simulink model "launch_gate_exp"  (R2022b)
settings: Solver=FixedStepDiscrete  StartTime=0.0  StopTime=5  FixedStep=0.001  RelTol=1e-3
InitFcn:
  | if ~exist('P','var') || ~isfield(P,'gate_version'), P=gate_params(launch_tcs_params()); end
model workspace (MAT data in the model file):
  w_2 : Simulink.Parameter (value not decoded)
undefined symbols (not defined in the file): A, a, B, b, C, D, DiscIntNeverNeededParam, Iz, K, k1, K1, k2, K2, L1, L2, m, magnitude, Phi, Sample_time, Steer_Ratio
libraries: simulink x26, slpidlib x13, Solver_SF x1, dsparch4 x1
(part 6 of 7)

== matlab function launch_gate_exp/牵引效率计算/右前轮 ==
  data: Tw input; Fx_est output; omega_meas input; Fz input; Fx_raw output; Fx_limited output; omega_hat_out output; e_omega output; wv output
function [Fx_est, Fx_raw, Fx_limited, omega_hat_out, e_omega, wv] = ...
    FrontWheelFxObserver(Tw, omega_meas, Fz)

%#codegen
% 单轮纵向驱动力观测器
% 输入仅保留时变信号：
%   Tw         : 轮端驱动力矩 [N*m]
%   omega_meas : 实测车轮角速度 [rad/s]
%   Fz         : 单轮垂直载荷 [N]
%
% 输出：
%   Fx_est        : 最终纵向驱动力估计 [N]
%   Fx_raw        : 原始观测力估计 [N]
%   Fx_limited    : 限幅后力估计 [N]
%   omega_hat_out : 观测器内部估计轮速 [rad/s]
%   e_omega       : 轮速误差 [rad/s]
%   wv            : 低速平滑权重 [-]

% =========================================================
% 1. 固定参数区：根据具体车轮统一在这里调整
% =========================================================

Re = 0.834;              % 有效滚动半径 [m]
Jw = 110.64;            % 车轮等效转动惯量 [kg*m^2]
Ts = 0.001;             % 采样周期 [s]

mu = 0.7;               % 等效附着系数 [-]

l_omega = 50.0;         % 轮速误差反馈增益
fF = 3.0;               % 轮胎力观测带宽 [Hz]
gamma_F = Jw / Re * (2*pi*fF)^2;

enable_smc = 0;         % 是否启用滑模鲁棒项：1启用，0关闭
phi = 1.5;              % 滑模边界层厚度 [rad/s]
Func_ratio = 0.10;      % 未建模力比例，建议0.05~0.20
ks = Re / Jw * Func_ratio * mu * max(Fz, 0.0);

enable_lpf = 0;         % 是否启用输出低通：1启用，0关闭
tau_F = 0.08;           % 输出低通时间常数 [s]

v0 = 0.10;              % 低速权重起点 [m/s]
v1 = 0.80;              % 低速权重终点 [m/s]

eps_neg = 0.0;          % 允许负驱动力比例；严格驱动力估计取0
T_offset = 0.0;         % 轮端扭矩零偏 [N*m]
T_dead = 10.0;          % 扭矩死区 [N*m]

allow_brake_force = 0;  % 0：只估计驱动力；1：允许估计制动力

% =========================================================
% 2. 持久状态变量
% =========================================================

persistent omega_hat
persistent Fx_hat
persistent Fx_filt
persistent initialized

if isempty(initialized)
    omega_hat = 0.0;
    Fx_hat = 0.0;
    Fx_filt = 0.0;
    initialized = false;
end

if ~initialized
    omega_hat = omega_meas;
    Fx_hat = 0.0;
    Fx_filt = 0.0;
    initialized = true;
end

% =========================================================
% 3. 参数保护
% =========================================================

Jw_safe = max(Jw, 1e-6);
Re_safe = max(Re, 1e-6);
Ts_safe = max(Ts, 1e-6);
phi_safe = max(phi, 1e-6);
tau_safe = max(tau_F, Ts_safe);

Fz_safe = max(Fz, 0.0);
mu_safe = max(mu, 0.0);

if v1 <= v0
    v1_safe = v0 + 1e-3;
else
    v1_safe = v1;
end

% =========================================================
% 4. 扭矩零偏与死区处理
% =========================================================

Tw_corr = Tw - T_offset;

if abs(Tw_corr) < T_dead
    Tw_eff = 0.0;
else
    if Tw_corr > 0.0
        Tw_eff = Tw_corr - T_dead;
    else
        Tw_eff = Tw_corr + T_dead;
    end
end

if allow_brake_force < 0.5
    if Tw_eff < 0.0
        Tw_eff = 0.0;
    end
end

% =========================================================
% 5. 轮速误差
% =========================================================

e_omega = omega_meas - omega_hat;

% =========================================================
% 6. 滑模鲁棒项
% =========================================================

s = e_omega / phi_safe;

if s > 1.0
    sat_s = 1.0;
elseif s < -1.0
    sat_s = -1.0;
else
    sat_s = s;
end

if enable_smc > 0.5
    smc_term = ks * sat_s;
else
    smc_term = 0.0;
end

% =========================================================
% 7. 观测器状态更新
% =========================================================
%
% omega_hat_dot = Tw/Jw - Re/Jw*Fx_hat + l_omega*e_omega + ks*sat(e/phi)
% Fx_hat_dot    = -gamma_F*e_omega

omega_hat_dot = ...
    Tw_eff / Jw_safe ...
    - Re_safe / Jw_safe * Fx_hat ...
    + l_omega * e_omega ...
    + smc_term;

Fx_hat_dot = -gamma_F * e_omega;

omega_hat = omega_hat + Ts_safe * omega_hat_dot;
Fx_hat = Fx_hat + Ts_safe * Fx_hat_dot;

% =========================================================
% 8. 物理限幅与抗积分发散
% =========================================================

Fx_max = mu_safe * Fz_safe;

if allow_brake_force > 0.5
    Fx_min = -mu_safe * Fz_safe;
else
    Fx_min = -eps_neg * Fz_safe;
end

if Fx_hat > Fx_max
    Fx_hat = Fx_max;
elseif Fx_hat < Fx_min
    Fx_hat = Fx_min;
end

Fx_raw = Fx_hat;

if Fx_raw > Fx_max
    Fx_limited = Fx_max;
elseif Fx_raw < Fx_min
    Fx_limited = Fx_min;
else
    Fx_limited = Fx_raw;
end

% =========================================================
% 9. 低速平滑权重
% =========================================================

vw = abs(Re_safe * omega_meas);

wv = (vw - v0) / (v1_safe - v0);

if wv > 1.0
    wv = 1.0;
elseif wv < 0.0
    wv = 0.0;
end

wv = wv * wv * (3.0 - 2.0 * wv);

Fx_weighted = wv * Fx_limited;

% =========================================================
% 10. 输出低通滤波
% =========================================================

if enable_lpf > 0.5
    alpha = exp(-Ts_safe / tau_safe);
    Fx_filt = alpha * Fx_filt + (1.0 - alpha) * Fx_weighted;
    Fx_est = Fx_filt;
else
    Fx_filt = Fx_weighted;
    Fx_est = Fx_weighted;
end

omega_hat_out = omega_hat;

end

== matlab function launch_gate_exp/驱动防滑模块/MATLAB Function3 ==
  data: vfl input; v output; vfr input; vrl input; vrr input; omega input; brk input; st input
function v = fcn(vfl,vfr,vrl,vrr,omega,brk,st)
d = 2.36;
brk_bank = 40;
st_bank = 10;

v = 0;
if abs(st) <= st_bank && brk < brk_bank
    v = min([vfl,vfr,vrl,vrr]);
elseif abs(st) <= st_bank && brk >= brk_bank
    v = max([vfl,vfr,vrl,vrr]);
elseif abs(st) > st_bank && brk >= brk_bank
    v = 0.5*max([vfl+vrl-d*omega,vfr+vrr+d*omega]);
elseif abs(st) > st_bank && brk < brk_bank
    v = 0.5*max([vfl+vrl-d*omega,vfr+vrr+d*omega]);
end

== matlab function launch_gate_exp/牵引效率计算/左前轮 ==
  data: Tw input; Fx_est output; omega_meas input; Fz input; Fx_raw output; Fx_limited output; omega_hat_out output; e_omega output; wv output
function [Fx_est, Fx_raw, Fx_limited, omega_hat_out, e_omega, wv] = ...
    FrontWheelFxObserver(Tw, omega_meas, Fz)

%#codegen
% 单轮纵向驱动力观测器
% 输入仅保留时变信号：
%   Tw         : 轮端驱动力矩 [N*m]
%   omega_meas : 实测车轮角速度 [rad/s]
%   Fz         : 单轮垂直载荷 [N]
%
% 输出：
%   Fx_est        : 最终纵向驱动力估计 [N]
%   Fx_raw        : 原始观测力估计 [N]
%   Fx_limited    : 限幅后力估计 [N]
%   omega_hat_out : 观测器内部估计轮速 [rad/s]
%   e_omega       : 轮速误差 [rad/s]
%   wv            : 低速平滑权重 [-]

% =========================================================
% 1. 固定参数区：根据具体车轮统一在这里调整
% =========================================================

Re = 0.834;              % 有效滚动半径 [m]
Jw = 110.64;            % 车轮等效转动惯量 [kg*m^2]
Ts = 0.001;             % 采样周期 [s]

mu = 0.7;               % 等效附着系数 [-]

l_omega = 50.0;         % 轮速误差反馈增益
fF = 3.0;               % 轮胎力观测带宽 [Hz]
gamma_F = Jw / Re * (2*pi*fF)^2;

enable_smc = 0;         % 是否启用滑模鲁棒项：1启用，0关闭
phi = 1.5;              % 滑模边界层厚度 [rad/s]
Func_ratio = 0.10;      % 未建模力比例，建议0.05~0.20
ks = Re / Jw * Func_ratio * mu * max(Fz, 0.0);

enable_lpf = 0;         % 是否启用输出低通：1启用，0关闭
tau_F = 0.08;           % 输出低通时间常数 [s]

v0 = 0.10;              % 低速权重起点 [m/s]
v1 = 0.80;              % 低速权重终点 [m/s]

eps_neg = 0.0;          % 允许负驱动力比例；严格驱动力估计取0
T_offset = 0.0;         % 轮端扭矩零偏 [N*m]
T_dead = 10.0;          % 扭矩死区 [N*m]

allow_brake_force = 0;  % 0：只估计驱动力；1：允许估计制动力

% =========================================================
% 2. 持久状态变量
% =========================================================

persistent omega_hat
persistent Fx_hat
persistent Fx_filt
persistent initialized

if isempty(initialized)
    omega_hat = 0.0;
    Fx_hat = 0.0;
    Fx_filt = 0.0;
    initialized = false;
end

if ~initialized
    omega_hat = omega_meas;
    Fx_hat = 0.0;
    Fx_filt = 0.0;
    initialized = true;
end

% =========================================================
% 3. 参数保护
% =========================================================

Jw_safe = max(Jw, 1e-6);
Re_safe = max(Re, 1e-6);
Ts_safe = max(Ts, 1e-6);
phi_safe = max(phi, 1e-6);
tau_safe = max(tau_F, Ts_safe);

Fz_safe = max(Fz, 0.0);
mu_safe = max(mu, 0.0);

if v1 <= v0
    v1_safe = v0 + 1e-3;
else
    v1_safe = v1;
end

% =========================================================
% 4. 扭矩零偏与死区处理
% =========================================================

Tw_corr = Tw - T_offset;

if abs(Tw_corr) < T_dead
    Tw_eff = 0.0;
else
    if Tw_corr > 0.0
        Tw_eff = Tw_corr - T_dead;
    else
        Tw_eff = Tw_corr + T_dead;
    end
end

if allow_brake_force < 0.5
    if Tw_eff < 0.0
        Tw_eff = 0.0;
    end
end

% =========================================================
% 5. 轮速误差
% =========================================================

e_omega = omega_meas - omega_hat;

% =========================================================
% 6. 滑模鲁棒项
% =========================================================

s = e_omega / phi_safe;

if s > 1.0
    sat_s = 1.0;
elseif s < -1.0
    sat_s = -1.0;
else
    sat_s = s;
end

if enable_smc > 0.5
    smc_term = ks * sat_s;
else
    smc_term = 0.0;
end

% =========================================================
% 7. 观测器状态更新
% =========================================================
%
% omega_hat_dot = Tw/Jw - Re/Jw*Fx_hat + l_omega*e_omega + ks*sat(e/phi)
% Fx_hat_dot    = -gamma_F*e_omega

omega_hat_dot = ...
    Tw_eff / Jw_safe ...
    - Re_safe / Jw_safe * Fx_hat ...
    + l_omega * e_omega ...
    + smc_term;

Fx_hat_dot = -gamma_F * e_omega;

omega_hat = omega_hat + Ts_safe * omega_hat_dot;
Fx_hat = Fx_hat + Ts_safe * Fx_hat_dot;

% =========================================================
% 8. 物理限幅与抗积分发散
% =========================================================

Fx_max = mu_safe * Fz_safe;

if allow_brake_force > 0.5
    Fx_min = -mu_safe * Fz_safe;
else
    Fx_min = -eps_neg * Fz_safe;
end

if Fx_hat > Fx_max
    Fx_hat = Fx_max;
elseif Fx_hat < Fx_min
    Fx_hat = Fx_min;
end

Fx_raw = Fx_hat;

if Fx_raw > Fx_max
    Fx_limited = Fx_max;
elseif Fx_raw < Fx_min
    Fx_limited = Fx_min;
else
    Fx_limited = Fx_raw;
end

% =========================================================
% 9. 低速平滑权重
% =========================================================

vw = abs(Re_safe * omega_meas);

wv = (vw - v0) / (v1_safe - v0);

if wv > 1.0
    wv = 1.0;
elseif wv < 0.0
    wv = 0.0;
end

wv = wv * wv * (3.0 - 2.0 * wv);

Fx_weighted = wv * Fx_limited;

% =========================================================
% 10. 输出低通滤波
% =========================================================

if enable_lpf > 0.5
    alpha = exp(-Ts_safe / tau_safe);
    Fx_filt = alpha * Fx_filt + (1.0 - alpha) * Fx_weighted;
    Fx_est = Fx_filt;
else
    Fx_filt = Fx_weighted;
    Fx_est = Fx_weighted;
end

omega_hat_out = omega_hat;

end

== matlab function launch_gate_exp/质心侧偏角滑模观测器估计/Subsystem/MATLAB Function ==
  data: vx input; d_vy_model output; delta_f input; vy_hat input; gamma_hat input; d_gamma_model output
function [d_vy_model, d_gamma_model] = fcn(vx, delta_f, vy_hat, gamma_hat)

% 声明我们将使用来自MATLAB基础工作区的参数
m = 18530;%质量
Iz = 67536;%绕Z轴的转动惯量
a = 2.043;%前轴距
b=1.362;%后轴距
% Cf = 1360400;%前侧偏刚度
% Cr = 1611200;%后侧偏刚度
 Cf = 304828*2;Cr = 417040*2; % 仿真用

% 防止vx为0导致计算错误
if abs(vx) < 0.1
    vx = 0.1;
end

% 二自由度模型方程
d_vy_model = (-(Cf + Cr) / (m * vx)) * vy_hat + ...
             ((b * Cr - a * Cf) / (m * vx) - vx) * gamma_hat + ...
             (Cf / m) * delta_f;

d_gamma_model = ((b * Cr - a * Cf) / (Iz * vx)) * vy_hat - ...
                ((a^2 * Cf + b^2 * Cr) / (Iz * vx)) * gamma_hat + ...
                (a * Cf / Iz) * delta_f;

== matlab function launch_gate_exp/质心侧偏角滑模观测器估计/Subsystem1/MATLAB Function ==
  data: vx input; d_vy_model output; delta_f input; vy_hat input; gamma_hat input; d_gamma_model output
function [d_vy_model, d_gamma_model] = fcn(vx, delta_f, vy_hat, gamma_hat)

% 声明我们将使用来自MATLAB基础工作区的参数
m = 18530;%质量
Iz = 67536;%绕Z轴的转动惯量
a = 2.043;%前轴距
b=1.362;%后轴距
Cf = 1360400;%前侧偏刚度
Cr = 1611200;%后侧偏刚度

% 防止vx为0导致计算错误
if abs(vx) < 0.1
    vx = 0.1;
end

% 二自由度模型方程
d_vy_model = (-(Cf + Cr) / (m * vx)) * vy_hat + ...
             ((b * Cr - a * Cf) / (m * vx) - vx) * gamma_hat + ...
             (Cf / m) * delta_f;

d_gamma_model = ((b * Cr - a * Cf) / (Iz * vx)) * vy_hat - ...
                ((a^2 * Cf + b^2 * Cr) / (Iz * vx)) * gamma_hat + ...
                (a * Cf / Iz) * delta_f;

== matlab function launch_gate_exp/PF车速估计 ==
  data: ax_m input; vx_est output; ay_m input; r_m input; vy_est output; init_vx input; init_vy input
function [vx_est, vy_est] = fcn_ImprovedPF(ax_m, ay_m, r_m, init_vx, init_vy)
% 基于改进粒子滤波的车速估计
% 严格按照论文公式 (5)-(19) 实现

% --- 参数定义 (可根据实际情况调整) ---
persistent particles weights first_run
persistent T mx my mr Q R

if isempty(first_run)
    % 初始化参数
    N = 200; % 粒子数量 (论文伪代码步骤 0)
    T = 0.01; % 采样时间，对应传感器更新频率 (0.01s)
    
    % 自定义常数 (公式 17) - 需要根据调试确定
    mx = 0.5; 
    my = 0.5;
    mr = 0.1;
    
    % 过程噪声标准差 (公式 12 & 18) - 这里的 u 对应 xi
    sigma_proc = [0.1; 0.1; 0.01]; % [xi_x, xi_y, xi_z]
    Q = diag(sigma_proc.^2); 

    % 观测噪声标准差 (公式 13)
    sigma_meas = [0.2; 0.2; 0.01]; % [omega_ax, omega_ay, omega_r]
    R = diag(sigma_meas.^2);
    
    % --- 1. 初始化滤波器 (论文伪代码步骤 1) ---
    % 状态向量 X = [vx, ax, vy, ay, r]' (5维)
    % 粒子初始化：在初始值附近添加随机扰动
    particles = zeros(5, N);
    particles(1, :) = init_vx + randn(1, N) * 0.5; % vx
    particles(2, :) = ax_m + randn(1, N) * 0.1;    % ax
    particles(3, :) = init_vy + randn(1, N) * 0.1; % vy
    particles(4, :) = ay_m + randn(1, N) * 0.1;    % ay
    particles(5, :) = r_m + randn(1, N) * 0.01;    % r
    
    weights = ones(1, N) / N; % 初始化权重
    
    first_run = 0;
end

N = size(particles, 2);
particles_next = zeros(5, N);

% 测量向量 Z_k (公式 13上方定义)
Z_k = [ax_m; ay_m; r_m]; 

% --- 2. 粒子滤波主循环 ---
% 对应论文伪代码的步骤 2-8 (针对每个时刻)

% 预计算 G 矩阵的一部分 (公式 11) 和 L 矩阵的一部分 (公式 17)
% 注意：G 和 L 实际上在每个粒子计算中略有不同吗？
% 论文中 G 是常数矩阵，但 L 取决于测量值与上一时刻状态的差，
% 且公式 (19) X_k = F*X_k-1 + P_k + G*L*xi
% 这里我们需要对每个粒子进行循环

for i = 1:N
    % 提取第 i 个粒子上一时刻的状态 X_k-1
    X_prev = particles(:, i);
    vx_prev = X_prev(1);
    ax_prev = X_prev(2);
    vy_prev = X_prev(3);
    ay_prev = X_prev(4);
    r_prev  = X_prev(5);
    
    % --- 计算状态转移矩阵 F_k (公式 10) ---
    % 注意：原论文公式(10)中有笔误，第二行和第四行应该是全0行还是保持加速度不变？
    % 通常 CA (Constant Acceleration) 模型加速度导数为0。
    % 论文公式(10) F_k 矩阵：
    % Row 1: vx = vx + ax*T + vy*r*T (源自 ax = vx_dot - vy*r -> vx_dot = ax + vy*r) -> 离散化: vx_k = vx_k-1 + ax_k-1*T + vy_k-1*r_k-1*T (对应公式 7)
    % Row 2: ax = ax (常数模型) -> 0 1 0 0 0
    % Row 3: vy = vy + ay*T - vx*r*T (源自 ay = vy_dot + vx*r -> vy_dot = ay - vx*r) -> 离散化: vy_k = vy_k-1 + ay_k-1*T - vx_k-1*r_k-1*T (对应公式 8)
    % Row 4: ay = ay -> 0 0 0 1 0
    % Row 5: r = r -> 0 0 0 0 1
    
    F_k = [1, T,  r_prev*T, 0, 0;
           0, 1,         0, 0, 0;
          -r_prev*T, 0,  1, T, 0;
           0, 0,         0, 1, 0;
           0, 0,         0, 0, 1];
       
    % --- 3. 计算提议分布修正项 P_k (公式 14) ---
    % 论文中 a_x,k-1 是粒子状态，而 Z 中的 a_x 是当前测量值。
    % 公式 (14) 利用了测量值与粒子状态的差值。
    % 注意下标：公式里用的是 k-1 时刻的测量值和粒子，但在实时运行中，我们通常拿当前测量值去修正预测。
    % 也就是论文提到的 "基于 k-1 时刻传感器测量值...与 k-1 时刻每个粒子的...差值"。
    % 这里为了代码简洁，假设输入的 ax_m 即为 k-1 时刻（或者当前时刻用来修正前一步）。
    % 严格照公式：
    diff_ax = ax_m - ax_prev; % (a_xz,k-1 - a^i_x,k-1)
    diff_ay = ay_m - ay_prev; % (a_yz,k-1 - a^i_y,k-1)
    diff_r  = r_m  - r_prev;  % (r_z,k-1 - r^i_k-1)
    
    P_k = [T * (diff_ax + diff_r); % 第一行对应 vx 的修正
           diff_ax;                % 第二行对应 ax 的修正
           T * (diff_ay + diff_r); % 第三行对应 vy 的修正
           diff_ay;                % 第四行对应 ay 的修正
           diff_r];                % 第五行对应 r  的修正
           
    % --- 计算自适应增益矩阵 L_k (公式 17) ---
    L_k = [mx * diff_ax, 0, 0;
           0, my * diff_ay, 0;
           0, 0, mr * diff_r];
       
    % --- 计算过程噪声矩阵 G (公式 11) ---
    G = [T^2/2, 0, 0;
         T,     0, 0;
         0, T^2/2, 0;
         0, T,     0;
         0, 0,     T];
         
    % --- 生成标准高斯噪声 xi (公式 18) ---
    % xi 对应伪代码中的 "相互独立的标准高斯噪声"
    xi = randn(3, 1); 
    
    % --- 4. 状态预测 (公式 19) ---
    % X_k = F_k * X_k-1 + P_k + G * L_k * xi
    particles_next(:, i) = F_k * X_prev + P_k + G * L_k * xi;
    
    % --- 5. 权重更新 (伪代码步骤 6 & 7) ---
    % 计算该粒子的预测观测值 Z_pre (公式 13)
    % Z = [ax, ay, r]'
    % 状态向量 X = [vx, ax, vy, ay, r]' -> 对应的索引是 2, 4, 5
    Z_pre = [particles_next(2, i); 
             particles_next(4, i); 
             particles_next(5, i)];
         
    % 计算似然 (高斯分布)
    % likelihood = (1/sqrt((2*pi)^3 * det(R))) * exp(-0.5 * (Z_k - Z_pre)' * inv(R) * (Z_k - Z_pre));
    % 简化计算 (忽略常数项，因为最后会归一化)
    error = Z_k - Z_pre;
    likelihood = exp(-0.5 * (error' / R * error));
    
    weights(i) = weights(i) * likelihood;
end

% --- 6. 权重归一化 (伪代码步骤 10) ---
sum_weights = sum(weights);
if sum_weights > 0
    weights = weights / sum_weights;
else
    weights = ones(1, N) / N; % 防止除以零
end

% --- 7. 重采样 (伪代码步骤 9) ---
% 有效粒子数 (N_eff) 判断是否需要重采样
N_eff = 1 / sum(weights.^2);
if N_eff < N / 2
    particles_next = Resample(particles_next, weights, N);
    weights = ones(1, N) / N;
end

% 更新粒子集
particles = particles_next;

% --- 8. 输出状态估计 (伪代码步骤 11) ---
% 加权平均
vx_est = sum(particles(1, :) .* weights);
vy_est = sum(particles(3, :) .* weights);

end

% --- 辅助函数：重采样 (Systematic Resampling) ---
function new_particles = Resample(particles, weights, N)
    cdf = cumsum(weights);
    new_particles = zeros(size(particles));
    u = rand / N;
    j = 1;
    for i = 1:N
        u_i = u + (i - 1) / N;
        while u_i > cdf(j)
            j = j + 1;
            if j > N, j = N; end
        end
        new_particles(:, i) = particles(:, j);
    end
end

== matlab function launch_gate_exp/加速度滑模观测/MATLAB Function ==
  data: gamma_m input; phi_est output; phi_GPS input; GPS_valid input; gamma_corrected output; e_gamma_est output
function [phi_est, gamma_corrected, e_gamma_est] = GPS_INS_SlidingMode(gamma_m, phi_GPS, GPS_valid)
%% GPS/INS融合 - 滑模观测器
% 输入:
%   gamma_m   - INS测量的横摆角速度 (rad/s)
%   phi_GPS   - GPS测量的航向角 (rad)
%   GPS_valid - GPS数据有效标志
% 输出:
%   phi_est         - 估计的航向角 (rad)
%   gamma_corrected - 校正后的横摆角速度 (rad/s)
%   e_gamma_est     - 估计的横摆角速度偏差 (rad/s)

%% 参数设置
persistent phi_hat e_gamma_hat phi_GPS_last initialized

dt_sim = 0.001;      % 仿真步长 (s)

% ===== 滑模增益（主要调参对象）=====
k1 = 5;              % 航向角校正增益
k2 = 0.5;            % 角速度偏差校正增益
lambda = 10;         % 滑模面斜率

% 边界层厚度（消除抖振）
epsilon = 0.01;      % 越小越精确，但抖振越大

%% 初始化
if isempty(initialized)
    phi_hat = 0;
    e_gamma_hat = 0;
    phi_GPS_last = 0;
    initialized = true;
end

%% 滑模观测器核心算法

% 状态方程：
% phi_dot = gamma_m - e_gamma（真实角速度 = 测量值 - 偏差）
% e_gamma_dot ≈ 0（偏差缓慢变化）

if GPS_valid
    % 滑模面：s = phi_GPS - phi_hat
    s = phi_GPS - phi_hat;
    
    % 饱和函数（替代sign函数，减少抖振）
    if abs(s) > epsilon
        sat_s = sign(s);
    else
        sat_s = s / epsilon;
    end
    
    % 滑模观测器方程
    % 航向角估计
    phi_hat_dot = (gamma_m - e_gamma_hat) + k1 * sat_s;
    
    % 角速度偏差估计（利用滑模的等效控制）
    e_gamma_hat_dot = -k2 * sat_s;
    
    % 积分更新
    phi_hat = phi_hat + phi_hat_dot * dt_sim;
    e_gamma_hat = e_gamma_hat + e_gamma_hat_dot * dt_sim;
    
    % 保存GPS值
    phi_GPS_last = phi_GPS;
    
else
    % GPS无效时，纯惯性推算
    phi_hat = phi_hat + (gamma_m - e_gamma_hat) * dt_sim;
    % e_gamma_hat 保持不变
end

%% 输出
phi_est = phi_hat;
e_gamma_est = e_gamma_hat;
gamma_corrected = gamma_m - e_gamma_hat;

end

== matlab function launch_gate_exp/加速度滑模观测/MATLAB Function1 ==
  data: a_xm input; a_xc output; a_ym input; v_xGPS input; v_yGPS input; gamma_c input; GPS_update_flag input; a_yc output; e_ax_est output; e_ay_est output; reset input
function [a_xc, a_yc, e_ax_est, e_ay_est] = accel_SMO_correction(a_xm, a_ym, v_xGPS, v_yGPS, gamma_c, GPS_update_flag, reset)
% 加速度滑模观测器校正
% 输入：
%   a_xm, a_ym      - INS测量的加速度 (m/s^2)
%   v_xGPS, v_yGPS  - GPS测量的速度 (m/s)
%   gamma_c         - 校正后的横摆角速度 (rad/s)
%   GPS_update_flag - GPS更新标志 (1=有新数据)
%   reset           - 复位信号
% 输出：
%   a_xc, a_yc      - 校正后的加速度
%   e_ax_est, e_ay_est - 估计的加速度偏差

% 采样时间
dt = 0.001;     % 仿真步长
DT = 0.05;      % GPS采样周期

% 滑模观测器增益（需根据实际调参）
persistent k1 k2 lambda1 lambda2
if isempty(k1)
    k1 = 5;       % 速度误差增益
    k2 = 5;
    lambda1 = 0.5; % 加速度偏差增益
    lambda2 = 0.5;
end

% 持久变量（状态记忆）
persistent v_xI v_yI e_ax e_ay initialized
persistent a_xm_sum a_ym_sum sum_count

if isempty(initialized) || reset
    v_xI = 0;      % INS积分速度 x
    v_yI = 0;      % INS积分速度 y
    e_ax = 0;      % 加速度偏差估计 x
    e_ay = 0;      % 加速度偏差估计 y
    a_xm_sum = 0;  % 加速度累加（用于GPS周期内求和）
    a_ym_sum = 0;
    sum_count = 0;
    initialized = true;
end

% 累加加速度（对应论文中的求和项）
a_xm_sum = a_xm_sum + a_xm;
a_ym_sum = a_ym_sum + a_ym;
sum_count = sum_count + 1;

% 速度积分（考虑横摆角速度耦合，对应式3-10）
% v_xI(k+1) = v_xI(k) + dt*a_xm + DT*(v_yI*gamma_c - e_ax - n_ax)
% 简化：每步用校正后的加速度积分
a_xc_temp = a_xm - e_ax;
a_yc_temp = a_ym - e_ay;

% 考虑横摆角速度耦合的速度更新
v_xI = v_xI + dt * (a_xc_temp + v_yI * gamma_c);
v_yI = v_yI + dt * (a_yc_temp - v_xI * gamma_c);

% GPS更新时刻：执行滑模校正
if GPS_update_flag == 1
    % 速度误差（观测残差）
    e_vx = v_xI - v_xGPS;
    e_vy = v_yI - v_yGPS;
    
    % 滑模切换函数
    s_x = sign(e_vx);
    s_y = sign(e_vy);
    
    % 也可用饱和函数避免抖振
    % epsilon = 0.1;
    % s_x = sat_func(e_vx, epsilon);
    % s_y = sat_func(e_vy, epsilon);
    
    % 速度校正（直接用GPS速度重置，或软校正）
    % 软校正方式：
    v_xI = v_xI - k1 * DT * s_x;
    v_yI = v_yI - k2 * DT * s_y;
    
    % 加速度偏差更新（滑模观测器核心）
    e_ax = e_ax + lambda1 * DT * s_x;
    e_ay = e_ay + lambda2 * DT * s_y;
    
    % 限幅防止发散
    e_ax = max(min(e_ax, 2), -2);
    e_ay = max(min(e_ay, 2), -2);
    
    % 清零累加器
    a_xm_sum = 0;
    a_ym_sum = 0;
    sum_count = 0;
end

% 输出校正后的加速度（式3-12）
a_xc = a_xm - e_ax;
a_yc = a_ym - e_ay;

% 输出偏差估计（用于调试）
e_ax_est = e_ax;
e_ay_est = e_ay;

end

% 饱和函数（可选，减少抖振）
function y = sat_func(x, epsilon)
    if abs(x) <= epsilon
        y = x / epsilon;
    else
        y = sign(x);
    end
end

== matlab function launch_gate_exp/质心侧偏角观测/MATLAB Function ==
  data: x_hat input; x_dot output; u input; z_meas input; z_hat output
function [x_dot, z_hat] = fcn(x_hat, u, z_meas)

    % === 车辆物理参数 ===
    mv = 18530;       % Vehicle total mass (kg)
    Izz = 67536;      % Second moment of mass (kg m^2)
    L1 = 2.043;        % CG to front axle (m)
    L2 = 1.362;        % CG to rear axle (m)
    Cf1 = 304828 * 2;     % Front cornering stiffness (N/rad) - 对应图中 C_F\delta^1
    Cf2 = 417040 * 2;     % Rear cornering stiffness (N/rad) - 对应图中 C_F\delta^2

    % === 观测器参数===
    Lambda = [100, 0;    % 增益矩阵 (3x2)
          0, 100;    
          0, 1000];   
    lambda_param = 1;
    Ts = 0.001;           % 离散采样时间 (Discrete Sample Time)

    % === 1. 解包状态变量和输入 ===
    % x_hat = [Vg_est; delta_est; r_est] 
    x1 = x_hat(1); % V_G
    x2 = x_hat(2); % delta (侧偏角)
    x3 = x_hat(3); % psi_dot (横摆角速度)

    % u = [beta; Fl1; Fl2]
    u1 = u(1); % beta
    u2 = u(2); % Fl1
    u3 = u(3); % Fl2
    
    % 防止分母为0
    if abs(x1) < 0.1
        x1 = 0.1; 
    end

    % === 2. 计算估计的输出 z_hat  ===
    % z = [Vg; psi_dot]
    h_NL = [x1; x3]; 
    z_hat = h_NL;

    % === 3. 计算观测误差 (z - z_hat) ===
    error = z_meas - z_hat;

    % === 4. 计算 Sign_eq 函数 ===
    sign_term = (2/pi) * atan(lambda_param * error);

    % === 5. 计算非线性函数 ===
    term1_1 = (1/mv) * (u2 * cos(x2 - u1) + u3 * cos(x2));
    term1_2 = (1/mv) * Cf2 * (-x2 + L2*x3/x1) * sin(x2);
    term1_3 = (1/mv) * Cf1 * (u1 - x2 - L1*x3/x1) * sin(x2 - u1);
    
    dx1_val = term1_1 + term1_2 + term1_3;

    term2_1 = 1/(mv*x1) * (u2 * sin(u1 - x2) - u3 * sin(x2)) ;
    term2_2 = 1/(mv*x1) * Cf1 * (u1 - x2 - L1*x3/x1) * cos(u1 - x2);
    term2_3 = 1/(mv*x1) * Cf2 * (-x2 + L2*x3/x1) * cos(x2) - x3;
    
    dx2_val = term2_1 + term2_2 + term2_3;

    term3_1 = (1/Izz) * ( L1 * u2 * sin(u1) - L2 * Cf2 * (-x2 + L2*x3/x1) ); 
    term3_2 = (1/Izz) * L1 * Cf1 * (u1 - x2 - L1*x3/x1) * cos(u1);
    
    dx3_val = term3_1 + term3_2;
    
    f_NL = [dx1_val; dx2_val; dx3_val];

    % === 6. 最终观测器状态导数 ===
    % x_hat_dot = f_NL(x_hat, u) + Lambda * sign_eq(z - z_hat)
    x_dot = f_NL + Lambda * sign_term;
end

== matlab function launch_gate_exp/软土扭矩分配/牵引功率目标计算 ==
  data: dt_s input; drawbar_power_w output; wheel_omegas_radps input; previous_applied_torques_n_m input; longitudinal_speed_mps input; implement_force_x_n input; wheel_power_w output; phi_raw output; filtered_phi output; filtered_normalized_phi output; lambda_est output; objective_valid output
function [drawbar_power_w, wheel_power_w, phi_raw, filtered_phi, filtered_normalized_phi, lambda_est, objective_valid] = MF_TractionEfficiencyObjective(dt_s, wheel_omegas_radps, previous_applied_torques_n_m, longitudinal_speed_mps, implement_force_x_n)

% 牵引效率目标函数计算模块
%
% 本模块计算牵引效率相关的在线优化目标：
% eta = P_drawbar / P_wheel
%
% 并构造 Dinkelbach 差值型目标：
% phi = P_drawbar - lambda * P_wheel

persistent has_filtered_power filtered_drawbar_power_state filtered_wheel_power_state
persistent has_filtered_phi filtered_phi_state filtered_normalized_phi_state
persistent lambda_state

if isempty(has_filtered_power)

    has_filtered_power = 0.0;
    filtered_drawbar_power_state = 0.0;
    filtered_wheel_power_state = 0.0;

    has_filtered_phi = 0.0;
    filtered_phi_state = 0.0;
    filtered_normalized_phi_state = 0.0;

    lambda_state = 0.0;
end

%% 输入整理

dt = max(double(dt_s), 0.0);
omegas = row4_local(wheel_omegas_radps);
applied_torques = row4_local(previous_applied_torques_n_m);

vx = double(longitudinal_speed_mps);
implement_force = double(implement_force_x_n);

%% 轮端输入功率计算

% 轮端输入功率 P_wheel = sum(T_i * omega_i)。
% 只保留非负驱动功率，避免制动功率或异常信号影响牵引效率评价。
wheel_drive_powers = zeros(1, 4);

for index = 1:4
    wheel_drive_powers(index) = max(0.0, applied_torques(index) * abs(omegas(index)));
end

wheel_power_w = sum(wheel_drive_powers);

%% 有效牵引功率计算

% 农具阻力方向通常与车辆行驶方向相反。
% 前进时，如果 implement_force 为负，则 -implement_force 为有效牵引阻力。
% 倒车时符号相反。
if vx > 0.08
    drawbar_force = max(0.0, -implement_force);
elseif vx < -0.08
    drawbar_force = max(0.0, implement_force);
else
    drawbar_force = 0.0;
end

drawbar_power_w = drawbar_force * abs(vx);

%% 目标函数有效性判断

% 轮端输入功率过低或车速过低时，牵引效率计算不可靠。
objective_valid = wheel_power_w >= 100.0 && abs(vx) > 0.08;

%% 功率滤波

alpha_objective = first_order_alpha_local(dt, 0.7);

if has_filtered_power <= 0.5 || ~objective_valid

    filtered_drawbar_power_state = drawbar_power_w;
    filtered_wheel_power_state = wheel_power_w;
    has_filtered_power = 1.0;

else

    filtered_drawbar_power_state = filtered_drawbar_power_state + ...
        alpha_objective * (drawbar_power_w - filtered_drawbar_power_state);

    filtered_wheel_power_state = filtered_wheel_power_state + ...
        alpha_objective * (wheel_power_w - filtered_wheel_power_state);

    has_filtered_power = 1.0;
end

%% lambda 牵引效率参数更新

if objective_valid

    eta_instant = drawbar_power_w / max(wheel_power_w, 1.0e-9);

    alpha_lambda = first_order_alpha_local(dt, 1.0);

    lambda_state = lambda_state + alpha_lambda * (eta_instant - lambda_state);
end

lambda_est = lambda_state;

%% Dinkelbach 差值型性能指标

phi_raw = drawbar_power_w - lambda_est * wheel_power_w;

% 归一化性能指标，用于降低功率量级变化对极值寻优的影响。
normalized_phi = phi_raw / max(abs(wheel_power_w), 1000.0);

%% 性能指标滤波

if has_filtered_phi <= 0.5 || ~objective_valid

    filtered_phi_state = phi_raw;
    filtered_normalized_phi_state = normalized_phi;
    has_filtered_phi = 1.0;

else

    filtered_phi_state = filtered_phi_state + ...
        alpha_objective * (phi_raw - filtered_phi_state);

    filtered_normalized_phi_state = filtered_normalized_phi_state + ...
        alpha_objective * (normalized_phi - filtered_normalized_phi_state);

    has_filtered_phi = 1.0;
end

filtered_phi = filtered_phi_state;
filtered_normalized_phi = filtered_normalized_phi_state;

end


function output = row4_local(values)

% 将输入信号整理为 1×4 行向量。

input_values = double(values);
output = zeros(1, 4);

for index = 1:4
    output(index) = input_values(index);
end

end


function alpha = first_order_alpha_local(dt, time_constant_s)

% 一阶低通滤波系数：
% y(k) = y(k-1) + alpha * [u(k) - y(k-1)]

if dt <= 0.0 || time_constant_s <= 0.0
    alpha = 1.0;
else
    alpha = dt / (time_constant_s + dt);
end

end

== matlab function launch_gate_exp/软土扭矩分配/四轮目标滑移率计算 ==
  data: current_time_s input; adaptive_targets output; dt_s input; filtered_normalized_phi input; objective_valid input; kappa_valid input; target_base_out output; gradient_estimates output
function [adaptive_targets, target_base_out, gradient_estimates] = MF_AdaptiveSlipTarget4W(current_time_s, dt_s, filtered_normalized_phi, objective_valid, kappa_valid)

% 四轮自适应目标滑移率生成模块
%
% 采用多变量极值寻优思想，对四个车轮的目标滑移率进行独立更新。
%
% 四轮顺序：
% 1：左前轮
% 2：右前轮
% 3：左后轮
% 4：右后轮

persistent target_base_state gradient_state

if isempty(target_base_state)

    % 初始目标滑移率仍保持原前后轴标定值。
    target_base_state = [0.078, 0.078, 0.128, 0.128];

    % 四轮梯度估计初值。
    gradient_state = zeros(1, 4);
end

%% 输入整理

time_s = double(current_time_s);
dt = max(double(dt_s), 0.0);
normalized_phi = double(filtered_normalized_phi);
valid_vec = row4_local(kappa_valid);

%% 极值寻优参数

% 四轮扰动频率，单位 Hz。
frequencies = [0.7, 0.9, 1.1, 1.3];

% 目标滑移率扰动幅值。
perturb_amp = 0.002;

% 目标滑移率基值自适应增益。
adapt_gain = 0.0006;

% 目标滑移率允许范围。
target_min = 0.03;
target_max = 0.25;

% 梯度低通滤波系数。
alpha_gradient = first_order_alpha_local(dt, 0.8);

%% 是否允许更新目标基值

update_enabled = double(objective_valid) > 0.5 && all(valid_vec > 0.5);

%% 生成四轮扰动信号

sine_signals = zeros(1, 4);

for index = 1:4
    sine_signals(index) = sin(2.0 * pi * frequencies(index) * time_s);
end

%% 梯度估计与目标基值更新

if update_enabled

    for index = 1:4

        % 极值寻优解调。
        % 性能指标与扰动信号相乘，用于估计该轮目标滑移率变化对牵引效率目标的边际影响。
        gradient_raw = 2.0 * normalized_phi * sine_signals(index) / perturb_amp;

        % 梯度估计低通滤波。
        gradient_state(index) = gradient_state(index) + ...
            alpha_gradient * (gradient_raw - gradient_state(index));

        % 限制每个采样周期目标滑移率基值的最大变化量。
        max_delta = 0.003 * dt;

        target_delta = clamp_local(adapt_gain * gradient_state(index) * dt, -max_delta, max_delta);

        % 更新目标滑移率基值。
        target_base_state(index) = clamp_local(target_base_state(index) + target_delta, target_min, target_max);
    end
end

%% 输出四轮目标滑移率

adaptive_targets = zeros(1, 4);

for index = 1:4

    % 最终目标 = 基值 + 小幅正弦扰动。
    adaptive_targets(index) = clamp_local( ...
        target_base_state(index) + perturb_amp * sine_signals(index), ...
        target_min, target_max);
end

% 调试输出，可在 Simulink 中不连接。
target_base_out = target_base_state;
gradient_estimates = gradient_state;

end


function output = row4_local(values)

% 将输入信号整理为 1×4 行向量。

input_values = double(values);
output = zeros(1, 4);

for index = 1:4
    output(index) = input_values(index);
end

end


function alpha = first_order_alpha_local(dt, time_constant_s)

% 一阶低通滤波系数。

if dt <= 0.0 || time_constant_s <= 0.0
    alpha = 1.0;
else
    alpha = dt / (time_constant_s + dt);
end

end


function value = clamp_local(value_in, lower, upper)

% 数值限幅函数。

value = min(max(double(value_in), double(lower)), double(upper));

end

== matlab function launch_gate_exp/牵引效率计算/计算平均边际贡献 ==
  data: v_all input; phi output
function phi = shapley_calc(v_all)

% 输入:
% v_all: 16x1
%
% 子集顺序:
%
% 1  -> []
% 2  -> [1]
% 3  -> [2]
% 4  -> [3]
% 5  -> [4]
% 6  -> [1 2]
% 7  -> [1 3]
% 8  -> [1 4]
% 9  -> [2 3]
% 10 -> [2 4]
% 11 -> [3 4]
% 12 -> [1 2 3]
% 13 -> [1 2 4]
% 14 -> [1 3 4]
% 15 -> [2 3 4]
% 16 -> [1 2 3 4]
%
% 输出:
% phi = [FL; FR; RL; RR]

%% 平移法消除负值

v_min = min(v_all);

if v_min < 0
    v_all = v_all - v_min;
end

%% 参数

n = 4;

fact = factorial(0:n);

phi = zeros(4,1);

%% 联盟定义

coalitions = [...
    0 0 0 0;  % 1
    1 0 0 0;  % 2
    0 1 0 0;  % 3
    0 0 1 0;  % 4
    0 0 0 1;  % 5
    1 1 0 0;  % 6
    1 0 1 0;  % 7
    1 0 0 1;  % 8
    0 1 1 0;  % 9
    0 1 0 1;  % 10
    0 0 1 1;  % 11
    1 1 1 0;  % 12
    1 1 0 1;  % 13
    1 0 1 1;  % 14
    0 1 1 1;  % 15
    1 1 1 1]; % 16

%% Shapley计算

for i = 1:n

    for idx = 1:16

        S = coalitions(idx,:);

        % 若联盟中已有玩家i
        if S(i) == 1
            continue;
        end

        % 联盟大小
        k = sum(S);

        % 权重
        w = fact(k+1) * fact(n-k) / fact(n+1);

        % v(S)
        v_S = v_all(idx);

        % 构造 S∪{i}
        S_with_i = S;
        S_with_i(i) = 1;

        %% 查找 S∪{i} 对应索引

        idx_Si = 1;

        for j = 1:16

            if isequal(coalitions(j,:), S_with_i)

                idx_Si = j;
                break;

            end

        end

        % v(S∪{i})
        v_Si = v_all(idx_Si);

        % Shapley累加
        phi(i) = phi(i) + w * (v_Si - v_S);

    end

end

phi_min = min(phi);

if phi_min < 0
    phi = phi - phi_min;
end

end

== matlab function launch_gate_exp/协同博弈扭矩分配/MATLAB Function ==
  data: v input; alpha output
function alpha = fcn(v)

if v < 0.5
    alpha = 0;
elseif v < 5
    alpha = (v - 0.5)/(5 - 0.5);
else
    alpha = 1;
end

== matlab function launch_gate_exp/牵引效率计算/MATLAB Function3 ==
  data: Fx input; V_all output; Vx input; T input; uF input; mu input; Fz input; slip input; Mz_ref input; Traction_all output; lamdaN_all output; lamda_all output; Mz_all output
function [V_all,Traction_all,lamdaN_all,lamda_all,Mz_all] = shapley_value_all(...
Fx,...
Vx,...
T,...
uF,...
mu,...
Fz,...
slip,...
Mz_ref)

%% 参数

kf = 3;   % 前轮牵引权重
kr = 6;   % 后轮牵引权重

w1 = 100000;  % 滑转率损失权重
w2 = 5000;    % 附着利用率均衡权重
w3 = 0.0001;  % 横摆稳定损失权重

% 半轮距
bf = 2.39/2;
br = 2.33/2;

%% 初始化

V_all = zeros(16,1);
Traction_all = zeros(16,1);
lamdaN_all = zeros(16,1);
lamda_all = zeros(16,1);
Mz_all = zeros(16,1);

%% 16个联盟

coalitions = [...
    0 0 0 0;  % 空集-1
    1 0 0 0;  % 2
    0 1 0 0;  % 3
    0 0 1 0;  % 4
    0 0 0 1;  % 5
    1 1 0 0;  % 6
    1 0 1 0;  % 7
    1 0 0 1;  % 8
    0 1 1 0;  % 9
    0 1 0 1;  % 10
    0 0 1 1;  % 11
    1 1 1 0;  % 12
    1 1 0 1;  % 13
    1 0 1 1;  % 14
    0 1 1 1;  % 15
    1 1 1 1];  % 16

%% 遍历所有联盟

for k = 1:16

    coalition = coalitions(k,:)';

    %% 联盟数据

    Fx_s    = Fx    .* coalition;
    T_s     = T     .* coalition;
    uF_s    = uF   .* coalition;
    mu_s    = mu    .* coalition;
    Fz_s    = Fz    .* coalition;
    slip_s  = slip   .* coalition;

    %% 1 牵引能力项

    F_front = uF_s(1) + uF_s(2);
    F_rear  = uF_s(3) + uF_s(4);

    traction_term = ...
        kf * F_front + ...
        kr * F_rear;

    %% 2 滑转率损失

    
    % 只保留联盟中的驱动轮滑转率
    slip_active = abs(slip_s);

    % 防止空集导致 max([]) 问题
if sum(coalition) == 0

    lamdaN = 0;

else

    % 最大滑转率
    slip_max = max(slip_active);

    % 四次方强化惩罚
    lamdaN = slip_max^4;

end


    %% 3 附着利用率

    lambda_term = 0;

    for i = 1:4

        if coalition(i) == 1

            denom = uF_s(i);

            if abs(denom) > 1e-6

                lambda_i = Fx_s(i) / denom;

                % 平方强化
                lambda_term = ...
                    lambda_term + lambda_i^2;

            end

        end

    end

    %% 4 横摆力矩

    Mz = ...
        (-Fx_s(1) + Fx_s(2)) * bf + ...
        (-Fx_s(3) + Fx_s(4)) * br;

    %Mz = 

    %% 5 价值函数

    V_all(k) = ...
        traction_term ...
        - w1 * lamdaN ...
        + w2 * lambda_term ...
        - w3 * (Mz - Mz_ref)^2;

    Traction_all(k) = traction_term;
    lamdaN_all(k) = -w1 * lamdaN;
    lamda_all(k) = w2 * lambda_term;
    Mz_all(k) = - w3 * (Mz - Mz_ref)^2;

end

end

== matlab function launch_gate_exp/软土分配策略/MATLAB Function ==
  data: wheel_speeds_rpm input; selected_torques_n_m output; front_steer_angles_deg input; longitudinal_speed_mps input; applied_torques_n_m input; drive_torque_enabled input; baseline_torques_n_m input; wheel_torque_limits_n_m input; control_kappa output; filtered_kappa output; kappa_valid output; adaptive_targets output; cbf_torque_upper_bounds output; cbf_active output; nominal_torques_n_m output; soft_diag output
function [selected_torques_n_m, control_kappa, filtered_kappa, kappa_valid, adaptive_targets, cbf_torque_upper_bounds, cbf_active, nominal_torques_n_m, soft_diag] = shiche_soft_soil_adaptive_allocation(wheel_speeds_rpm, front_steer_angles_deg, longitudinal_speed_mps, applied_torques_n_m, drive_torque_enabled, baseline_torques_n_m, wheel_torque_limits_n_m)
%SHICHE_SOFT_SOIL_ADAPTIVE_ALLOCATION Real-vehicle soft-soil clamp allocator.
%
% MATLAB Function block version for VCU code generation. All numeric states,
% constants, intermediate arrays, and outputs are single precision.
%
% Wheel vector order is fixed as a 4x1 column:
%   [L1, R1, L2, R2] = [left-front, right-front, left-rear, right-rear]
%
% This block assumes an upstream load-based/basic four-wheel torque allocator
% already exists. baseline_torques_n_m is used as the reproducible anchor
% allocation. This real-vehicle version intentionally avoids QP, matrix solves,
% and active-set enumeration: it applies slip-tracking torque correction and
% then clamps each wheel by the CBF safety upper bound.
%
% Inputs:
%   wheel_speeds_rpm        single, 4x1 wheel speeds in rpm, [L1 R1 L2 R2].
%   front_steer_angles_deg  single, [Steer_L1 Steer_R1] in deg, or one scalar.
%   longitudinal_speed_mps  single, vehicle longitudinal speed in m/s.
%   applied_torques_n_m     single, 4x1 actual or one-step delayed applied wheel
%                           torques in N*m, [L1 R1 L2 R2].
%   drive_torque_enabled    single flag, >0.5 enables adaptive update and CBF.
%   baseline_torques_n_m    single, 4x1 upstream basic allocation in N*m.
%   wheel_torque_limits_n_m single, 4x1 nonnegative wheel torque limits in N*m.
%
% Outputs are single. kappa_valid and cbf_active are 0/1 single flags. soft_diag
% has 26 entries:
%   1:6   front target, rear target, simplified allocator status, total torque
%         reduction by CBF clamp, baseline total torque, selected total torque
%   7:10  filtered slip derivatives
%   11:14 slip input gains
%   15:18 slip disturbance estimates
%   19:22 disturbance margins
%   23:26 wheel surface speeds

persistent has_filtered filtered_state filtered_dot_state disturbance_state

if isempty(has_filtered)
    has_filtered = zeros(4, 1, 'single');
    filtered_state = zeros(4, 1, 'single');
    filtered_dot_state = zeros(4, 1, 'single');
    disturbance_state = zeros(4, 1, 'single');
end

dt = single(0.02);
wheel_speeds = column4_local(wheel_speeds_rpm);
front_steers = front_steer_pair_local(front_steer_angles_deg);
control_vx = single(longitudinal_speed_mps);
applied_torques = column4_local(applied_torques_n_m);
base_torques = column4_local(baseline_torques_n_m);
wheel_limits = column4_local(wheel_torque_limits_n_m);
drive_enabled = single(drive_torque_enabled) > single(0.5);

for index = 1:4
    wheel_limits(index) = max(single(0.0), wheel_limits(index));
    base_torques(index) = clamp_local(base_torques(index), single(0.0), wheel_limits(index));
end

[control_kappa, filtered_kappa, kappa_valid, dot_kappa, rolling_speeds, wheel_omegas, surface_speeds, has_filtered, filtered_state, filtered_dot_state] = ...
    update_slip_local(wheel_speeds, front_steers, control_vx, dt, has_filtered, filtered_state, filtered_dot_state);

front_target_base = single(0.078);
rear_target_base = single(0.128);
adaptive_targets = zeros(4, 1, 'single');
adaptive_targets(1) = front_target_base;
adaptive_targets(2) = front_target_base;
adaptive_targets(3) = rear_target_base;
adaptive_targets(4) = rear_target_base;

input_gains = input_gains_local(kappa_valid, rolling_speeds, wheel_omegas);
[disturbance_state, disturbance_margins] = update_disturbance_local(kappa_valid, dot_kappa, input_gains, applied_torques, dt, disturbance_state);

front_error = axle_slip_error_local(filtered_kappa, kappa_valid, adaptive_targets(1), 1);
rear_error = axle_slip_error_local(filtered_kappa, kappa_valid, adaptive_targets(3), 2);

nominal_torques_n_m = zeros(4, 1, 'single');
cbf_torque_upper_bounds = zeros(4, 1, 'single');
cbf_active = zeros(4, 1, 'single');
for index = 1:4
    gain = input_gains(index);
    if drive_enabled && kappa_valid(index) > single(0.5) && isfinite(gain)
        if index <= 2
            axle_error = front_error;
        else
            axle_error = rear_error;
        end
        torque_delta = clamp_local(-single(20500.0) * axle_error, -single(2600.0), single(2600.0));
        nominal = base_torques(index) + torque_delta;
    else
        nominal = base_torques(index);
    end
    nominal_torques_n_m(index) = clamp_local(nominal, single(0.0), wheel_limits(index));

    if drive_enabled && kappa_valid(index) > single(0.5) && isfinite(gain)
        upper = (single(15.0) * (single(0.25) - filtered_kappa(index)) - disturbance_state(index) - disturbance_margins(index)) / gain;
        if ~isfinite(upper)
            upper = wheel_limits(index);
        end
        upper = clamp_local(upper, single(0.0), wheel_limits(index));
    else
        upper = wheel_limits(index);
    end
    cbf_torque_upper_bounds(index) = upper;
    if upper < base_torques(index) - single(1.0e-6)
        cbf_active(index) = single(1.0);
    end
end

selected_torques_n_m = zeros(4, 1, 'single');
for index = 1:4
    selected_torques_n_m(index) = clamp_local(nominal_torques_n_m(index), single(0.0), cbf_torque_upper_bounds(index));
end

allocator_status = single(1.0);
total_torque_reduction = sum(nominal_torques_n_m - selected_torques_n_m);
baseline_total_torque = sum(base_torques);
selected_total_torque = sum(selected_torques_n_m);

soft_diag = zeros(26, 1, 'single');
soft_diag(1) = front_target_base;
soft_diag(2) = rear_target_base;
soft_diag(3) = allocator_status;
soft_diag(4) = total_torque_reduction;
soft_diag(5) = baseline_total_torque;
soft_diag(6) = selected_total_torque;
for index = 1:4
    soft_diag(6 + index) = dot_kappa(index);
    soft_diag(10 + index) = input_gains(index);
    soft_diag(14 + index) = disturbance_state(index);
    soft_diag(18 + index) = disturbance_margins(index);
    soft_diag(22 + index) = surface_speeds(index);
end
end

function [raw_kappa, filtered_kappa, valid, dot_kappa, rolling_speeds, omegas, surface_speeds, has_filtered_out, filtered_state_out, filtered_dot_out] = update_slip_local(wheel_speeds, front_steers, vx_mps, dt, has_filtered_in, filtered_state_in, filtered_dot_in)
rpm_to_rad = single(2.0) * single(pi) / single(60.0);
radii = zeros(4, 1, 'single');
radii(1) = single(0.834);
radii(2) = single(0.834);
radii(3) = single(0.94);
radii(4) = single(0.94);
speed_abs = abs(single(vx_mps));
steer_l = front_steers(1) * single(pi) / single(180.0);
steer_r = front_steers(2) * single(pi) / single(180.0);
rolling_speeds = zeros(4, 1, 'single');
rolling_speeds(1) = abs(speed_abs * cos(steer_l));
rolling_speeds(2) = abs(speed_abs * cos(steer_r));
rolling_speeds(3) = speed_abs;
rolling_speeds(4) = speed_abs;
omegas = abs(single(wheel_speeds)) * rpm_to_rad;
surface_speeds = radii .* omegas;

raw_kappa = zeros(4, 1, 'single');
filtered_kappa = zeros(4, 1, 'single');
dot_kappa = zeros(4, 1, 'single');
valid = zeros(4, 1, 'single');
has_filtered_out = has_filtered_in;
filtered_state_out = filtered_state_in;
filtered_dot_out = filtered_dot_in;
for index = 1:4
    raw_kappa(index) = single(NaN);
    filtered_kappa(index) = single(NaN);
end

alpha_kappa = first_order_alpha_local(dt, single(0.04));
alpha_dot = first_order_alpha_local(dt, single(0.08));
for index = 1:4
    is_valid = speed_abs >= single(0.08) && surface_speeds(index) >= single(0.20) && isfinite(rolling_speeds(index)) && isfinite(surface_speeds(index));
    if is_valid
        valid(index) = single(1.0);
        raw_value = single(1.0) - rolling_speeds(index) / surface_speeds(index);
        raw_kappa(index) = clamp_local(raw_value, -single(1.0), single(1.0));
        if has_filtered_in(index) <= single(0.5) || ~isfinite(filtered_state_in(index))
            filtered_value = raw_kappa(index);
            raw_dot = single(0.0);
        else
            previous = filtered_state_in(index);
            filtered_value = previous + alpha_kappa * (raw_kappa(index) - previous);
            raw_dot = (filtered_value - previous) / dt;
        end
        filtered_dot_out(index) = filtered_dot_in(index) + alpha_dot * (raw_dot - filtered_dot_in(index));
        filtered_state_out(index) = filtered_value;
        has_filtered_out(index) = single(1.0);
        filtered_kappa(index) = filtered_value;
        dot_kappa(index) = filtered_dot_out(index);
    else
        if has_filtered_in(index) > single(0.5)
            raw_kappa(index) = filtered_state_in(index);
            filtered_kappa(index) = filtered_state_in(index);
        end
        filtered_dot_out(index) = single(0.0);
        dot_kappa(index) = single(0.0);
    end
end
end

function front_steers = front_steer_pair_local(front_steer_angles_deg)
% Accept [Steer_L1, Steer_R1] or one equivalent front-axle steer angle.
steer_input = single(front_steer_angles_deg);
front_steers = zeros(2, 1, 'single');
if numel(steer_input) >= 2
    front_steers(1) = steer_input(1);
    front_steers(2) = steer_input(2);
else
    front_steers(1) = steer_input(1);
    front_steers(2) = steer_input(1);
end
end

function gains = input_gains_local(valid, rolling_speeds, omegas)
radii = zeros(4, 1, 'single');
radii(1) = single(0.834);
radii(2) = single(0.834);
radii(3) = single(0.94);
radii(4) = single(0.94);
inertias = zeros(4, 1, 'single');
inertias(1) = single(450.0);
inertias(2) = single(450.0);
inertias(3) = single(650.0);
inertias(4) = single(650.0);
gains = zeros(4, 1, 'single');
for index = 1:4
    gains(index) = single(NaN);
end
for index = 1:4
    if valid(index) > single(0.5) && omegas(index) > single(0.0)
        gain = rolling_speeds(index) / (inertias(index) * radii(index) * omegas(index) * omegas(index));
        if gain >= single(1.0e-8)
            gains(index) = gain;
        end
    end
end
end

function [disturbance_out, margins] = update_disturbance_local(valid, dot_kappa, input_gains, applied_torques, dt, disturbance_in)
disturbance_out = disturbance_in;
margins = zeros(4, 1, 'single');
alpha_disturbance = first_order_alpha_local(dt, single(0.15));
for index = 1:4
    gain = input_gains(index);
    if valid(index) > single(0.5) && isfinite(gain)
        raw_estimate = dot_kappa(index) - gain * applied_torques(index);
        disturbance_out(index) = disturbance_in(index) + alpha_disturbance * (raw_estimate - disturbance_in(index));
        residual = raw_estimate - disturbance_out(index);
    else
        residual = single(0.0);
    end
    margins(index) = clamp_local(single(0.05) + single(0.05) * abs(residual), single(0.05), single(5.0));
end
end

function error = axle_slip_error_local(filtered_kappa, valid, target, axle_id)
total = single(0.0);
count = single(0.0);
if axle_id == 1
    start_index = 1;
    end_index = 2;
else
    start_index = 3;
    end_index = 4;
end
for index = start_index:end_index
    if valid(index) > single(0.5) && isfinite(filtered_kappa(index))
        total = total + filtered_kappa(index);
        count = count + single(1.0);
    end
end
if count > single(0.0)
    error = total / count - target;
else
    error = single(0.0);
end
end

function alpha = first_order_alpha_local(dt, time_constant_s)
if dt <= single(0.0) || time_constant_s <= single(0.0)
    alpha = single(1.0);
else
    alpha = dt / (time_constant_s + dt);
end
end

function value = clamp_local(value_in, lower, upper)
value = min(max(single(value_in), single(lower)), single(upper));
end

function output = column4_local(values)
input_values = single(values);
output = zeros(4, 1, 'single');
for index = 1:4
    output(index) = input_values(index);
end
end

== stateflow chart launch_gate_exp/总驱动力矩制定/负载工况_极限防抖 ==
  state Normal
    entry:
    T_hold = 0;
    during:
    T0_out = T0;
  state Limit_detect
    during:
    T0_out = T0;
  state Limit_hold
    entry:
    T_hold = T0;
    during:
    T_hold = T_hold + 0.02*(T0 - T_hold);
    T_hold = min(max(T_hold,2000),60000);
    T0_out = T_hold;
  (default) -> Normal
  Limit_detect -> Normal [order 1] : [(throttle < 0.7) || (load_rate < 0.9) || (abs(ax) > 0.1)]
  Normal -> Limit_detect : [(throttle > 0.8) && (load_rate > 0.9) && (abs(ax) < 0.1) ]
  Limit_hold -> Normal : [ (load_rate < 0.85) && (abs(ax) > 0.12)]
  Limit_detect -> Limit_hold [order 2] : [after(0.5,sec)]
  data: throttle input; ax input; Tmax input; load_rate input; T0 input; T0_out output; T_hold local; timer_start local

== matlab function launch_gate_exp/PID_Controller//直线循迹/MATLAB Function ==
  data: u input; y output
function y = lowpass_filter(u)
persistent prev_x prev_y;
if isempty(prev_x), prev_x = 0; end
if isempty(prev_y), prev_y = 0; end

% 差分方程: y(n) = 0.2452*u(n) + 0.2452*u(n-1) + 0.5095*y(n-1)
y = 0.2452*u + 0.2452*prev_x + 0.5095*prev_y;

% 更新状态
prev_x = double(u);
prev_y = double(y);
end
